simulink model "ETH01_Model"  (R2026b)
settings: Solver=FixedStepDiscrete  FixedStep=0.001
settings Model: Creator=lww  LastModifiedBy=lww
settings OptimizationCC: DefaultParameterBehavior=Inlined  DifferentSizesBufferReuse=on  EfficientTunableParamExpr=on  EnhancedBackFolding=on  OptimizationCustomize=off  OptimizeBlockOrder=speed  PassReuseOutputArgsAs=Individual arguments  RemoveInternalMemoryZeroInit=on  RemoveRootLevelIOMemoryZeroInit=on
settings DebuggingCC: ParameterTunabilityLossMsg=error
settings HardwareCC: ProdHWDeviceType=ARM Compatible->ARM Cortex-R  ProdLargestAtomicFloat=Double  ProdLargestAtomicInteger=Long
settings SFSimCC: MATLABDynamicMemAlloc=off
settings RTWCC: DataTypeReplacement=CDataTypesFixedWidth  Description=Embedded Coder  GenCodeOnly=on  GenerateReport=on  SystemTargetFile=ert.tlc  TemplateMakefile=ert_default_tmf
settings CodeAppCC: ForceParamTrailComments=on  IgnoreCustomStorageClasses=off  InsertBlockDesc=on  OperatorAnnotations=on  SFDataObjDesc=on  SimulinkDataObjDesc=on
settings ERTTargetCC: CombineSignalStateStructs=on  GenerateSampleERTMain=on  MaxIdInt16=INT16_MAX  MaxIdInt32=INT32_MAX  MaxIdInt64=INT64_MAX  MaxIdInt8=INT8_MAX  MaxIdUint16=UINT16_MAX  MaxIdUint32=UINT32_MAX  MaxIdUint64=UINT64_MAX  MaxIdUint8=UINT8_MAX  MinIdInt16=INT16_MIN  MinIdInt32=INT32_MIN  MinIdInt64=INT64_MIN  MinIdInt8=INT8_MIN

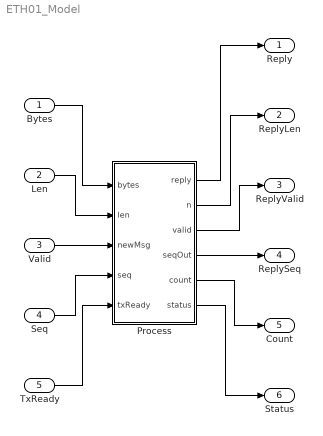
== system ETH01_Model ==
  Bytes : Inport  OutDataTypeStr=uint8  PortDimensions=256
  Len : Inport  Port=2  OutDataTypeStr=uint16
  Valid : Inport  Port=3  OutDataTypeStr=boolean
  Seq : Inport  Port=4  OutDataTypeStr=uint32
  TxReady : Inport  Port=5  OutDataTypeStr=boolean
  Process : MATLAB Function  TreatAsAtomicUnit=on
  Reply : Outport
  ReplyLen : Outport  Port=2
  ReplyValid : Outport  Port=3
  ReplySeq : Outport  Port=4
  Count : Outport  Port=5
  Status : Outport  Port=6
  wires:
  Process/6(status) -> Status/1
  Process/5(count) -> Count/1
  Process/4(seqOut) -> ReplySeq/1
  Process/3(valid) -> ReplyValid/1
  Process/2(n) -> ReplyLen/1
  Process/1(reply) -> Reply/1
  Bytes/1 -> Process/1(bytes)
  Len/1 -> Process/2(len)
  Valid/1 -> Process/3(newMsg)
  Seq/1 -> Process/4(seq)
  TxReady/1 -> Process/5(txReady)

== matlab function ETH01_Model/Process ==
  data: bytes input; reply output; len input; newMsg input; seq input; txReady input; n output; valid output; seqOut output; count output; status output
function [reply,n,valid,seqOut,count,status] = process(bytes,len,newMsg,seq,txReady)
%#codegen
persistent saved savedLen savedSeq pending handled
if isempty(pending)
 saved=zeros(256,1,'uint8'); savedLen=uint16(0); savedSeq=uint32(0); pending=false; handled=uint32(0);
end
reply=saved; n=savedLen; seqOut=savedSeq; valid=false; status=uint8(0);
if pending
 valid=true; status=uint8(2);
 if txReady, pending=false; end
elseif newMsg
 if len>256
  status=uint8(3);
 else
  saved=bytes;
  for k=1:256
   if k<=len, saved(k)=bitxor(bytes(k),uint8(90)); end
  end
  savedLen=len; savedSeq=seq; handled=handled+uint32(1); pending=true;
  reply=saved; n=savedLen; seqOut=savedSeq; valid=true; status=uint8(1);
  if txReady, pending=false; end
 end
end
count=handled;
end
